simulink model "wturbines"  (R2024b)
settings: Solver=ode4  StartTime=0.0  StopTime=inf  FixedStep=0.01  RelTol=1e-3
values from neighbouring files (symbols this model uses):
  A_k = 2E6    (= 2000000)    [initialize_turbine_parameters.m]
  air_density = 1.225    [initialize_turbine_parameters.m]
  alpha_pitch_exp = 0    [initialize_turbine_parameters.m]
  B_k = 1E4    (= 10000)    [initialize_turbine_parameters.m]
  brake_torque = 28116.2    [initialize_turbine_parameters.m]
  C_k = 0    [initialize_turbine_parameters.m]
  Cp_mat = nan(numel(tsr_vec), numel(pitch_vec))    [initialize_turbine_parameters.m]
  Cp_opt = 0.482    [initialize_turbine_parameters.m]
  Ct_mat = nan(size(Cp_mat))    [initialize_turbine_parameters.m]
  ctrl_mode = 1    [initialize_turbine_parameters.m]
  cut_in_wind_speed = 3.0    (= 3)    [initialize_turbine_parameters.m]
  cut_out_wind_speed = 25.0    (= 25)    [initialize_turbine_parameters.m]
  D_k = 0    [initialize_turbine_parameters.m]
  dr_mode = Simulink.Parameter(1)    [initialize_turbine_parameters.m]
  gearbox_ratio = 1    [initialize_turbine_parameters.m]
  generator_eff = 0.954    [initialize_turbine_parameters.m]
  inertia = 1.9E6    (= 1900000)    [initialize_turbine_parameters.m]
  K_i_gen = 1e2    (= 100)    [initialize_turbine_parameters.m]
  K_i_pitch = 0    [initialize_turbine_parameters.m]
  K_i_pitch_gs = 0    [initialize_turbine_parameters.m]
  K_omega_sq = 1/2 * (tsr_opt)^-3 * air_density * pi * (rotor_diameter / 2)^5 * Cp_opt / gearbox_ratio^3    (= 69831977.2177)    [initialize_turbine_parameters.m]
  K_p_gen = 1e2    (= 100)    [initialize_turbine_parameters.m]
  K_p_pitch = 1    [initialize_turbine_parameters.m]
  K_p_pitch_gs = 0.1    [initialize_turbine_parameters.m]
  max_gen_torque = 1.15 * rated_gen_torque    (= 35686440.711)    [initialize_turbine_parameters.m]
  MIN_ROT_SPEED = 1e-3    (= 0.001)    [initialize_turbine_parameters.m]
  Nt = 9    [init.m]
  pitch_all = T{:, col_pitch}    [initialize_turbine_parameters.m]
  pitch_rate_deg = 5    [initialize_turbine_parameters.m]
  pitch_vec = sort(pitch_vec(:))    [initialize_turbine_parameters.m]
  rated_power = 22E6    (= 22000000)    [initialize_turbine_parameters.m]
  rated_rotor_speed = 6.77    [initialize_turbine_parameters.m]
  rated_rotor_speed_rads = rated_rotor_speed * (2 * pi) / 60    (= 0.70895274216)    [initialize_turbine_parameters.m]
  rated_wind_speed = 11.0    (= 11)    [initialize_turbine_parameters.m]
  ROT_EMG_MAX_TOL = 1.15    [initialize_turbine_parameters.m]
  ROT_SPEED_MIN_TRANS = min_rotor_speed_rads    (= 0.19)    [initialize_turbine_parameters.m]
  ROT_SPEED_SP_DIFF = 0.1    [initialize_turbine_parameters.m]
  rotor_radius = rotor_diameter / 2    (= 142)    [initialize_turbine_parameters.m]
  rotor_speed_all = [0, rated_rotor_speed]    [initialize_turbine_parameters.m]
  rotor_speed_init = rotor_speed_init * (2 * pi) / 60    (= 1.25663706144)    [initialize_turbine_parameters.m]
  rotor_speed_ref_mode = 1    [initialize_turbine_parameters.m]
  tsr_opt = 9.153    [initialize_turbine_parameters.m]
  tsr_vec = sort(tsr_vec(:))    [initialize_turbine_parameters.m]
  u_all = T{:, col_u}    [initialize_turbine_parameters.m]
  u_rotor_speed_all = [cut_in_wind_speed, rated_wind_speed]    [initialize_turbine_parameters.m]
  yawing_rate = 5    [initialize_turbine_parameters.m]
undefined symbols (not defined in the file or in its folder): op_mode, turbineDataBytes
libraries: simulink x24, simulink_extras x14, slpidlib x8, slrealtimeiplib x4, svdutilitieslib x2, slctrl_autotuning x2, etargetslib x2, dspstat3 x1
(part 3 of 3)

== system wturbines/For Each Subsystem/Turbine Dynamics + Controller1/Control logic/Power controller/Lio downregulation/Pitch controller ==
  ws(t) : Inport
  ws_dr(t) : Inport  Port=2
  e_ω(t) : Inport  Port=3
  Constant : Constant  Value=0
  Derating : Switch  Criteria=u2 > Threshold  SaturateOnIntegerOverflow=off  InputSameDT=off
  PI controller : slpidlib/PID Controller  Controller=PI  Form=Parallel  TimeDomain=Continuous-time  UseExternalTs=off  SampleTime=-1  IntegratorMethod=Forward Euler  FilterMethod=Forward Euler  ControllerParametersSource=internal  P=K_p_pitch  I=K_i_pitch  UseKiTs=off  D=0  UseExternalDerivativeSource=off  N=100  UseFilter=on  TunerSelectOption=Transfer Function Based (PID Tuner App)  InitialConditionSource=internal  InitialConditionForIntegrator=0  InitialConditionForFilter=0  DifferentiatorICPrevScaledInput=0  ExternalReset=none  TrackingMode=off  Kt=1  LimitOutput=off  SatLimitsSource=internal  UpperSaturationLimit=inf  LowerSaturationLimit=-inf  LinearizeAsGain=on  AntiWindupMode=none  Kb=1  LimitIntegrator=off  UpperIntegratorSaturationLimit=inf  LowerIntegratorSaturationLimit=-inf  POutMin=[]  POutMax=[]  IOutMin=[]  IOutMax=[]  DOutMin=[]  DOutMax=[]  NOutMin=[]  NOutMax=[]  SumOutMin=[]  SumOutMax=[]  SaturationOutMin=[]  SaturationOutMax=[]  PParamMin=[]  PParamMax=[]  IParamMin=[]  IParamMax=[]  DParamMin=[]  DParamMax=[]  NParamMin=[]  NParamMax=[]  KbParamMin=[]  KbParamMax=[]  KtParamMin=[]  KtParamMax=[]  KbOutMin=[]  KbOutMax=[]  KtOutMin=[]  KtOutMax=[]  IntegratorOutMin=[]  IntegratorOutMax=[]  FilterOutMin=[]  FilterOutMax=[]  SumI1OutMin=[]  SumI1OutMax=[]  SumI2OutMin=[]  SumI2OutMax=[]  SumI3OutMin=[]  SumI3OutMax=[]  SumI4OutMin=[]  SumI4OutMax=[]  SumDOutMin=[]  SumDOutMax=[]  DifferentiatorOutMin=[]  DifferentiatorOutMax=[]  FilterDiffOutCoefMin=[]  FilterDiffOutCoefMax=[]  ReciprocalOutMin=[]  ReciprocalOutMax=[]  SumDenOutMin=[]  SumDenOutMax=[]  SumNumOutMin=[]  SumNumOutMax=[]  DivideOutMin=[]  DivideOutMax=[]  UdiffTsProdOutMin=[]  UdiffTsProdOutMax=[]  NTsProdOutMin=[]  NTsProdOutMax=[]  UintegralTsProdOutMin=[]  UintegralTsProdOutMax=[]  UngainTsProdOutMin=[]  UngainTsProdOutMax=[]  ClampingZeroOutDataTypeStr=Inherit: Inherit via back propagation  ClampingZeroOutMin=[]  ClampingZeroOutMax=[]  FilterDenConstantOutDataTypeStr=Inherit: Inherit via back propagation  FilterDenConstantOutMin=[]  FilterDenConstantOutMax=[]  PCopyOutDataTypeStr=Inherit: Inherit via back propagation  PCopyOutMin=[]  PCopyOutMax=[]  NCopyOutDataTypeStr=Inherit: Inherit via back propagation  NCopyOutMin=[]  NCopyOutMax=[]  IntegratorContinuousStateAttributes=''  IntegratorStateMustResolveToSignalObject=off  IntegratorRTWStateStorageClass=Auto  FilterContinuousStateAttributes=''  FilterStateMustResolveToSignalObject=off  FilterRTWStateStorageClass=Auto  ParallelPVariant=InternalParameters  IdealPVariant=Disabled  IVariant=InternalParameters  DVariant=Disabled  IntegratorVariant=Continuous  SatVariant=Disabled  AWVariant=Passthrough  PCopyVariant=Disabled  TRVariant=Disabled  FdbkBlocksVariant=Forward  IdealPFdbkVariant=Disabled  SatFdbkVariant=Disabled  DerivativeFilterVariant=Disabled  NVariant=Disabled  NCopyVariant=Disabled_SignalSpec  FilterICVariant=Disabled  IntegratorICVariant=InternalICs  ExternalResetVariant=Disabled  TRSumVariant=Passthrough  SumFdbkVariant=Disabled  SumVariant=Sum_PI  TsampFilterVariant=InternalTs  TsampNgainVariant=Passthrough  TsampIntegralVariant=Disabled_SignalSpec  ExternalSaturationOutDataTypeStr=Inherit: Same as second input  DerivativeSourceVariant=Disabled  PreIntVariant=InternalPreInt
  Sum : Sum  Inputs=-+|
  β(t) : Outport
  wires:
  Derating/1 -> β(t)/1
  ws_dr(t)/1 -> Sum/2
  ws(t)/1 -> Sum/1
  Sum/1 -> Derating/2  "(ws_dr - ws)(t)"
  e_ω(t)/1 -> PI controller/1
  Constant/1 -> Derating/1
  PI controller/1 -> Derating/3

== system wturbines/For Each Subsystem/Turbine Dynamics + Controller1/Control logic/Power controller/Lio downregulation/Torque controller ==
  ω_set(t) : Inport
  ws(t) : Inport  Port=2
  ws_dr(t) : Inport  Port=3
  e_ω(t) : Inport  Port=4
  P_set(t) : Inport  Port=5
  Derating : Switch  Criteria=u2 > Threshold  SaturateOnIntegerOverflow=off  InputSameDT=off
  Divide : Product  Inputs=*/
  Gain : Gain  Gain=1/gearbox_ratio
  PI controller : slpidlib/PID Controller  Controller=PI  Form=Parallel  TimeDomain=Continuous-time  UseExternalTs=off  SampleTime=-1  IntegratorMethod=Forward Euler  FilterMethod=Forward Euler  ControllerParametersSource=internal  P=K_p_gen  I=K_i_gen  UseKiTs=off  D=0  UseExternalDerivativeSource=off  N=100  UseFilter=on  TunerSelectOption=Transfer Function Based (PID Tuner App)  InitialConditionSource=internal  InitialConditionForIntegrator=0  InitialConditionForFilter=0  DifferentiatorICPrevScaledInput=0  ExternalReset=none  TrackingMode=off  Kt=1  LimitOutput=off  SatLimitsSource=internal  UpperSaturationLimit=inf  LowerSaturationLimit=-inf  LinearizeAsGain=on  AntiWindupMode=none  Kb=1  LimitIntegrator=off  UpperIntegratorSaturationLimit=inf  LowerIntegratorSaturationLimit=-inf  POutMin=[]  POutMax=[]  IOutMin=[]  IOutMax=[]  DOutMin=[]  DOutMax=[]  NOutMin=[]  NOutMax=[]  SumOutMin=[]  SumOutMax=[]  SaturationOutMin=[]  SaturationOutMax=[]  PParamMin=[]  PParamMax=[]  IParamMin=[]  IParamMax=[]  DParamMin=[]  DParamMax=[]  NParamMin=[]  NParamMax=[]  KbParamMin=[]  KbParamMax=[]  KtParamMin=[]  KtParamMax=[]  KbOutMin=[]  KbOutMax=[]  KtOutMin=[]  KtOutMax=[]  IntegratorOutMin=[]  IntegratorOutMax=[]  FilterOutMin=[]  FilterOutMax=[]  SumI1OutMin=[]  SumI1OutMax=[]  SumI2OutMin=[]  SumI2OutMax=[]  SumI3OutMin=[]  SumI3OutMax=[]  SumI4OutMin=[]  SumI4OutMax=[]  SumDOutMin=[]  SumDOutMax=[]  DifferentiatorOutMin=[]  DifferentiatorOutMax=[]  FilterDiffOutCoefMin=[]  FilterDiffOutCoefMax=[]  ReciprocalOutMin=[]  ReciprocalOutMax=[]  SumDenOutMin=[]  SumDenOutMax=[]  SumNumOutMin=[]  SumNumOutMax=[]  DivideOutMin=[]  DivideOutMax=[]  UdiffTsProdOutMin=[]  UdiffTsProdOutMax=[]  NTsProdOutMin=[]  NTsProdOutMax=[]  UintegralTsProdOutMin=[]  UintegralTsProdOutMax=[]  UngainTsProdOutMin=[]  UngainTsProdOutMax=[]  ClampingZeroOutDataTypeStr=Inherit: Inherit via back propagation  ClampingZeroOutMin=[]  ClampingZeroOutMax=[]  FilterDenConstantOutDataTypeStr=Inherit: Inherit via back propagation  FilterDenConstantOutMin=[]  FilterDenConstantOutMax=[]  PCopyOutDataTypeStr=Inherit: Inherit via back propagation  PCopyOutMin=[]  PCopyOutMax=[]  NCopyOutDataTypeStr=Inherit: Inherit via back propagation  NCopyOutMin=[]  NCopyOutMax=[]  IntegratorContinuousStateAttributes=''  IntegratorStateMustResolveToSignalObject=off  IntegratorRTWStateStorageClass=Auto  FilterContinuousStateAttributes=''  FilterStateMustResolveToSignalObject=off  FilterRTWStateStorageClass=Auto  ParallelPVariant=InternalParameters  IdealPVariant=Disabled  IVariant=InternalParameters  DVariant=Disabled  IntegratorVariant=Continuous  SatVariant=Disabled  AWVariant=Passthrough  PCopyVariant=Disabled  TRVariant=Disabled  FdbkBlocksVariant=Forward  IdealPFdbkVariant=Disabled  SatFdbkVariant=Disabled  DerivativeFilterVariant=Disabled  NVariant=Disabled  NCopyVariant=Disabled_SignalSpec  FilterICVariant=Disabled  IntegratorICVariant=InternalICs  ExternalResetVariant=Disabled  TRSumVariant=Passthrough  SumFdbkVariant=Disabled  SumVariant=Sum_PI  TsampFilterVariant=InternalTs  TsampNgainVariant=Passthrough  TsampIntegralVariant=Disabled_SignalSpec  ExternalSaturationOutDataTypeStr=Inherit: Same as second input  DerivativeSourceVariant=Disabled  PreIntVariant=InternalPreInt
  Sum : Sum  Inputs=-+|
  T_g(t) : Outport
  wires:
  Sum/1 -> Derating/2  "(ws_dr - ws)(t)"
  ws_dr(t)/1 -> Sum/2
  e_ω(t)/1 -> PI controller/1
  ws(t)/1 -> Sum/1
  Derating/1 -> T_g(t)/1
  P_set(t)/1 -> Divide/1
  ω_set(t)/1 -> Divide/2
  PI controller/1 -> Derating/1
  Divide/1 -> Gain/1
  Gain/1 -> Derating/3

== system wturbines/For Each Subsystem/Turbine Dynamics + Controller1/Control logic/Power controller/Lio downregulation/rads2rpm ==
  rad/s : Inport
  Multiply : Gain  Gain=1 / (2 * pi)
  Multiply1 : Gain  Gain=60
  rpm : Outport
  wires:
  Multiply/1 -> Multiply1/1
  rad/s/1 -> Multiply/1
  Multiply1/1 -> rpm/1

== system wturbines/For Each Subsystem/Turbine Dynamics + Controller1/Control logic/Power controller/ROSCO/Pitch controller ==
  ω_g(t) : Inport
  Δω_g(t) : Inport  Port=2
  β_min(t) : Inport  Port=3
  Constant : Constant  Value=rated_rotor_speed
  Gain : Gain  Gain=gearbox_ratio
  β(t) : Outport
  wires:
  Constant/1 -> Gain/1
  Gain/1 -> ?  "ω_g,rated"

== system wturbines/For Each Subsystem/Turbine Dynamics + Controller1/Control logic/Power controller/ROSCO/Torque controller ==
  ω_g(t) : Inport
  ws(t) : Inport  Port=2
  Δω_g(t) : Inport  Port=3
  β(t) : Inport  Port=4
  T_g(t) : Outport

== system wturbines/For Each Subsystem/Turbine Dynamics + Controller1/Control logic/Power controller/Gain-scheduled H∞ control /Pitch controller/rad2deg ==
  rad : Inport
  Radians to Degrees : simulink_extras/Transformations/Radians to Degrees
  deg : Outport
  wires:
  rad/1 -> Radians to Degrees/1
  Radians to Degrees/1 -> deg/1

== system wturbines/For Each Subsystem/Turbine Dynamics + Controller1/Control logic/Power controller/Kω2 controller/Pitch controller/   ==
  rpm : Inport
  Multiply : Gain  Gain=2 * pi
  Multiply1 : Gain  Gain=1 / 60
  rad/s : Outport
  wires:
  Multiply/1 -> Multiply1/1
  rpm/1 -> Multiply/1
  Multiply1/1 -> rad/s/1

== system wturbines/For Each Subsystem/Turbine Dynamics + Controller1/Control logic/Power controller/Kω2 controller/Pitch controller/rad2deg ==
  deg : Inport
  Degrees to Radians : simulink_extras/Transformations/Degrees to Radians
  rad : Outport
  wires:
  deg/1 -> Degrees to Radians/1
  Degrees to Radians/1 -> rad/1

== stateflow chart wturbines/For Each Subsystem/Turbine Dynamics + Controller1/Control logic/Wind Turbine State Machine ==
  state power_production
  state starting_up
  state shutting_down
  state emergency_stop
  state parked
  power_production -> emergency_stop [order 2] : [estop]
  starting_up -> power_production [order 1] : [(ctrl_mode == 1 && rot_speed >= ROT_SPEED_MIN_TRANS) || (ctrl_mode == 2 && abs(rot_speed_sp - rot_speed) <= ROT_SPEED_SP_DIFF)]
  power_production -> shutting_down [order 1] : [(~enable && ~estop) || ws <= 0.5*cut_in_wind_speed || ws >= cut_out_wind_speed]
  power_production -> starting_up [order 3] : [rot_speed < 0.1*ROT_SPEED_MIN_TRANS]
  starting_up -> shutting_down [order 2] : [(~enable || estop) || ws <= 0.5*cut_in_wind_speed]
  shutting_down -> emergency_stop [order 1] : [estop]
  parked -> starting_up : [enable && ~estop && ws >= cut_in_wind_speed]
  emergency_stop -> parked : [rot_speed <= MIN_ROT_SPEED]
  shutting_down -> parked [order 2] : [rot_speed <= MIN_ROT_SPEED]
  (default) -> parked
  data: ws input; rot_speed input; enable input; estop input; cut_in_wind_speed parameter; cut_out_wind_speed parameter; rated_rotor_speed_rads parameter; MIN_ROT_SPEED parameter double; op_mode output Enum: op_mode; rot_speed_sp input; ctrl_mode input; ROT_SPEED_SP_DIFF parameter double; ROT_SPEED_MIN_TRANS parameter double; ROT_EMG_MAX_TOL parameter

== matlab function wturbines/For Each Subsystem/Turbine Dynamics + Controller1/Control logic/Orientation Setpoint Calculation ==
  data: wind_dir input; orientation output; yaw_offset input
function orientation = yaw2orientation(wind_dir, yaw_offset)

orientation = wind_dir - yaw_offset;

if orientation < -180 
    orientation = orientation + 360;
elseif orientation >= 180
    orientation = orientation - 360;
end

== matlab function wturbines/For Each Subsystem/Turbine Dynamics + Controller1/Control logic/MATLAB Function ==
  data: u input; y output
function y = deadband_zoh(u)
  persistent last_val;
  if isempty(last_val)
    last_val = u;
  end
  if abs(u - last_val) >= 5
    last_val = u;
  end
  y = last_val;
end

== matlab function wturbines/MATLAB Function ==
  data: u input Bus: loggingData; y output Bus: loggingDataVectors
function y = splitLoggingData(u)
%#codegen

N = numel(u);

y.Cp             = zeros(1,N);
y.Ct             = zeros(1,N);
y.GenSpd         = zeros(1,N);
y.OpMode         = repmat(op_mode(0), 1, N);   % adapt default enum value
y.OrientationSpt = zeros(1,N);
y.Pitch          = zeros(1,N);
y.PitchSpt       = zeros(1,N);
y.RotSpd         = zeros(1,N);
y.eCtrlMode      = zeros(1,N,'int32');
y.TBrake         = zeros(1,N);
y.TGen           = zeros(1,N);
y.Ta             = zeros(1,N);
y.WsEff          = zeros(1,N);
y.YawTrue        = zeros(1,N);
y.HorWdSpd       = zeros(1,N);
y.HorWdDir       = zeros(1,N);
y.bEnable        = false(1,N);
y.bStop          = false(1,N);
y.WSpt           = zeros(1,N);

for k = 1:N
    y.Cp(k)             = u(k).Cp;
    y.Ct(k)             = u(k).Ct;
    y.GenSpd(k)         = u(k).GenSpd;
    y.OpMode(k)         = u(k).OpMode;
    y.OrientationSpt(k) = u(k).OrientationSpt;
    y.Pitch(k)          = u(k).Pitch;
    y.PitchSpt(k)       = u(k).PitchSpt;
    y.RotSpd(k)         = u(k).RotSpd;
    y.eCtrlMode(k)      = u(k).eCtrlMode;
    y.TBrake(k)         = u(k).TBrake;
    y.TGen(k)           = u(k).TGen;
    y.Ta(k)             = u(k).Ta;
    y.WsEff(k)          = u(k).WsEff;
    y.YawTrue(k)        = u(k).YawTrue;
    y.HorWdSpd(k)       = u(k).HorWdSpd;
    y.HorWdDir(k)       = u(k).HorWdDir;
    y.bEnable(k)        = u(k).bEnable;
    y.bStop(k)          = u(k).bStop;
    y.WSpt(k)           = u(k).WSpt;
end

== matlab function wturbines/RX FlowField Conditions/Enabled Subsystem/ZoH nan filter2 ==
  data: w input; w_filtered output single; w_saved input; Nt parameter
function w_filtered = zoh_nan_filter(w, w_saved, Nt)

if all(w(:) == 0)
    for i = 1:Nt
        w(i,:) = 0;
    end
end

w_filtered = w;
nan_idx = isnan(w);
w_filtered(nan_idx) = w_saved(nan_idx);

end

== matlab function wturbines/For Each Subsystem/Turbine Dynamics + Controller/Subsystem/Orientation Setpoint Calculation ==
  data: wind_dir input; orientation output; yaw_offset input
function orientation = yaw2orientation(wind_dir, yaw_offset)

orientation = wind_dir - yaw_offset;

if orientation < 0 
    orientation = orientation + 360;
elseif orientation >= 360
    orientation = orientation - 360;
end

== matlab function wturbines/For Each Subsystem/Turbine Dynamics + Controller/Subsystem/True Yaw Offset ==
  data: wind_dir input; orientation input; yaw output
function yaw = orientation2yaw(wind_dir, orientation)

yaw = wind_dir - orientation;

if yaw > 180
    yaw = yaw - 360;
elseif yaw < -180
    yaw = yaw + 360;
end

== matlab function wturbines/For Each Subsystem/Turbine Dynamics + Controller/MATLAB Function2 ==
  data: wd input; wd_meas output
function wd_meas = wind_dir_meas(wd)

wd_meas = wd;

== matlab function wturbines/For Each Subsystem/Turbine Dynamics + Controller/MATLAB Function3 ==
  data: ws input; ws_meas output
function ws_meas = wind_speed_meas(ws)

ws_meas = ws;

== matlab function wturbines/For Each Subsystem/Turbine Dynamics + Controller/Subsystem/Meas Yaw Offset ==
  data: wind_dir input; orientation input; yaw output
function yaw = orientation2yaw(wind_dir, orientation)

yaw = wind_dir - orientation;

if yaw > 180
    yaw = yaw - 360;
elseif yaw < -180
    yaw = yaw + 360;
end

== matlab function wturbines/For Each Subsystem/Turbine Dynamics + Controller1/Turbine Dynamics/True Yaw Offset ==
  data: wind_dir input; orientation input; yaw output
function yaw = orientation2yaw(wind_dir, orientation)

yaw = wind_dir - orientation;

if yaw > 180
    yaw = yaw - 360;
elseif yaw < -180
    yaw = yaw +360;
end

== matlab function wturbines/RX FlowField Conditions/Enabled Subsystem/ZoH nan filter1 ==
  data: w input; w_filtered output single; w_saved input; Nt parameter
function w_filtered = zoh_nan_filter(w, w_saved, Nt)

if all(w(:) == 0)
    for i = 1:Nt
        w(i,:) = 10;
    end
end

w_filtered = w;
nan_idx = isnan(w);
w_filtered(nan_idx) = w_saved(nan_idx);

end
